simulink model "Task 2 – Battery Modeling"  (R2025b)
settings: Solver=ode23tb  StartTime=0.0  StopTime=35  RelTol=5e-3
model workspace (MAT data in the model file):
  Eng : object (value not decoded)
  Nmtr = 18.5
  SteerLim = 60
  TrackPoints = [-15 -12 -9 -6 -3 5.58745102111e-16 2.81978007367 5.36354042717 7.38228007367 8.67839071119 9.125 8.67839071119 ... (270 elements, 90x3)]
  Trans : object (value not decoded)
  Ts = 0.02
  VEH : object (value not decoded)
symbols that are objects in the model workspace (value not decoded): Eng, Trans, VEH
undefined symbols (not defined in the file or in its folder): BdyFrm, InertFrm
libraries: autolibsharedcoupling x11, simulink x9, sim3dlib x7, autolibutils x5, autolibshareddiff x5, sim3dautolib x3, vehdynlibtirecommon x3, sharedtransform x3, vehdynlibdriver x2, vehdynlibviscommon x2, vehdynlibtire x1, autolibmappedmotor x1
(part 2 of 4)

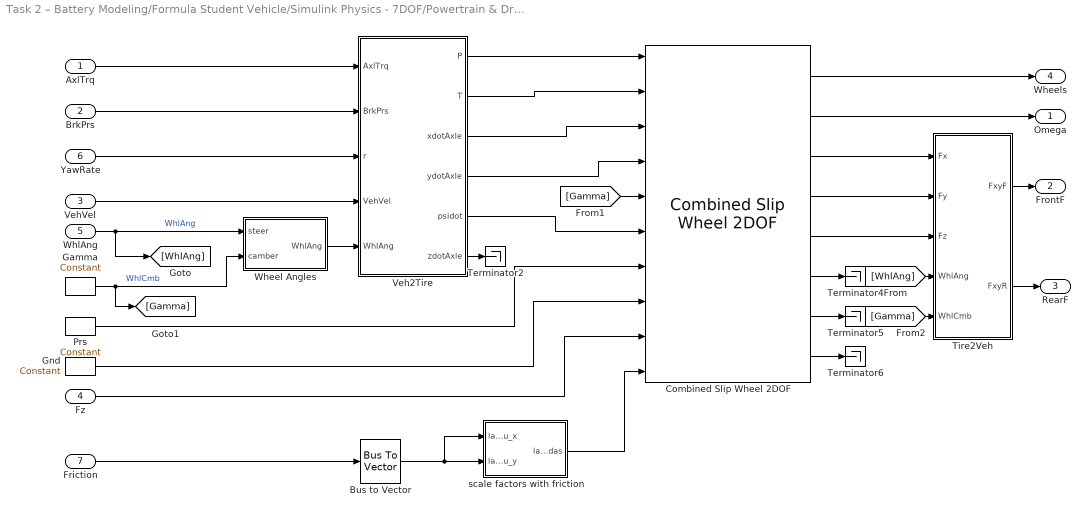
== system Task 2 – Battery Modeling/Formula Student Vehicle/Simulink Physics - 7DOF/Powertrain & Driveline/Brakes and Wheels ==
  AxlTrq : Inport
  BrkPrs : Inport  Port=2
  VehVel : Inport  Port=3
  Fz : Inport  Port=4  PortDimensions=4
  WhlAng : Inport  Port=5
  YawRate : Inport  Port=6
  Friction : Inport  Port=7
  Bus to Vector : BusToVector
  Combined Slip Wheel 2DOF : vehdynlibtire/Combined Slip Wheel 2DOF  tireType=External file  tireParamSet=skidpadtire.mat  vertType=None  plySteer=off  turnslip=off  BrakeType=Disc  mu_static=.3  mu_kinetic=.2  drum_abore=0.0508  drum_a=0.123  drum_c=0.212  drum_r=0.15  drum_theta1=0  drum_theta2=126  disk_abore=.05  Rm=.177  num_pads=2  brake_p_bpt=[1 11.4736842105263 21.9473684210526 32.4210526315789 42.8947368421053 53.3684210526316 63.8421052631579 74.3157894736842 84.7894736842105 95.2631578947368 105.736842105263 116.210526315789 126.684210526316 137.157894736842 147.631578947368 158.105263157895 168.578947368421 179.052631578947 189.526315789474 200]  brake_n_bpt=[0 52.6315789473684 105.263157894737 157.894736842105 210.526315789474 263.157894736842 315.789473684211 368.421052631579 421.052631578947 473.684210526316 526.315789473684 578.947368421053 631.578947368421 684.210526315789 736.842105263158 789.473684210526 842.105263157895 894.736842105263 947.368421052632 1000]  f_brake_t=[43.4900602404453 42.5056030554862 41.5350898940194 40.5780454442085 39.6340111501808 38.7025443887544 37.7832176914519 36.8756180088306 35.9793460143796 35.0940154454303 34.2192524787115 33.3546951383474 32.4999927342521 31.6548053290159 30.8188032315107 29.991666515561 29.1730845621415 28.362755623661 27.5603864089927 26.765691687993;498.991217495636 487.695866636631 476.560505099801 465.579679307235 454.748127933653 444.060772460445 433.51270824929 423.099196101319 412.81565427025 402.657650900201 392.620896861006 382.701238955775 372.894653477208 363.197240090814 353.605216024701 344.114910546964 334.722759712992 325.425301366216 316.219170376863 307.10109410434;954.492374750826 932.886130217776 911.585920305583 890.581313170261 869.862244717126 849.419000532136 829.242198807128 809.322774193808 789.651962526121 770.221286354971 751.0225412433 732.047782773203 713.289314220164 694.739674852612 676.391628817892 658.238154578366 640.272434863842 622.48784710877 604.877954344734 587.436496520688;1409.99353200602 1378.07639379892 1346.61133551136 1315.58294703329 1284.9763615006 1254.77722860383 1224.97168936497 1195.5463522863 1166.48827078199 1137.78492180974 1109.42418562559 1081.39432659063 1053.68397496312 1026.28210961441 999.178041611083 972.361398609768 945.822110014692 919.550392851325 893.536738312604 867.771898937035;1865.49468926121 1823.26665738007 1781.63675071715 1740.58458089631 1700.09047828407 1660.13545667552 1620.7011799228 1581.76993037878 1543.32457903786 1505.34855726451 1467.82583000789 1430.74087040806 1394.07863570608 1357.82454437621 1321.96445440427 1286.48464264117 1251.37178516554 1216.61293859388 1182.19552228048 1148.10730135338;2320.9958465164 2268.45692096121 2216.66216592293 2165.58621475934 2115.20459506754 2065.49368474721 2016.43067048064 1967.99350847127 1920.16088729373 1872.91219271928 1826.22747439018 1780.08741422549 1734.47329644903 1689.36697913801 1644.75086719747 1600.60788667257 1556.92146031639 1513.67548433643 1470.85430624835 1428.44270376973;2776.49700377159 2713.64718454235 2651.68758112871 2590.58784862237 2530.31871185102 2470.8519128189 2412.16016103848 2354.21708656376 2296.9971955496 2240.47582817405 2184.62911877248 2129.43395804292 2074.86795719199 2020.9094138998 1967.53727999066 1914.73113070398 1862.47113546724 1810.73803007899 1759.51309021622 1708.77810618608;3231.99816102678 3158.8374481235 3086.71299633449 3015.58948248539 2945.43282863449 2876.21014089059 2807.88965159632 2740.44066465625 2673.83350380547 2608.03946362882 2543.03076315477 2478.78050186034 2415.26261793494 2352.4518486616 2290.32369278385 2228.85437473538 2168.02081061809 2107.80057582154 2048.17187418409 1989.11350860242;3687.49931828197 3604.02771170464 3521.73841154027 3440.59111634842 3360.54694541796 3281.56836896228 3203.61914215416 3126.66424274874 3050.66981206134 2975.60309908359 2901.43240753707 2828.12704567777 2755.6572786779 2683.9942834234 2613.11010557704 2542.97761876678 2473.57048576894 2404.8631215641 2336.83065815196 2269.44891101877;4143.00047553716 4049.21797528579 3956.76382674606 3865.59275021144 3775.66106220143 3686.92659703397 3599.34863271199 3512.88782084123 3427.50612031721 3343.16673453836 3259.83405191936 3177.4735894952 3096.05193942085 3015.5367181852 2935.89651837023 2857.10086279818 2779.12016091979 2701.92566730665 2625.48944211983 2549.78431343512;4598.50163279235 4494.40823886693 4391.78924195184 4290.59438407447 4190.77517898491 4092.28482510566 3995.07812326983 3899.11139893372 3804.34242857308 3710.73036999313 3618.23569630166 3526.82013331263 3436.44660016381 3347.079152947 3258.68293116342 3171.22410682959 3084.66983607064 2998.98821304921 2914.1482260877 2830.11971585147;5054.00279004754 4939.59850244808 4826.81465715762 4715.59601793749 4605.88929576838 4497.64305317735 4390.80761382767 4285.3349770262 4181.17873682896 4078.2940054479 3976.63734068395 3876.16667713006 3776.84126090677 3678.62158770879 3581.46934395661 3485.34735086099 ...(+2764 chars)]  NOMPRES=78844.9  PRESMAX=99780  PRESMIN=45540  FNOMIN=866  FZMAX=1688  FZMIN=185  VXLOW=1  KPUMAX=0.165  KPUMIN=-0.179  ALPMAX=0.2338  ALPMIN=-0.2293  CAMMAX=0.0699  CAMMIN=-0.0699  LONGVL=10.23  FxRelFreqLwrLim=200*pi  FyRelFreqLwrLim=200*pi  MyRelFreqLwrLim=100*pi  omegao=0  UNLOADED_RADIUS=0.2667  WIDTH=0.2032  RIM_RADIUS=0.1651  ASPECT_RATIO=0.5  MASS=9.3  IYY=0.736  br=1e-3  GRAVITY=-9.81  zo=0  zdoto=0  BREFF=13.804  DREFF=1.08343  FREFF=0.16356  Q_RE0=0.9974  Q_V1=0.00077  Q_V2=9e-05  Q_FZ1=0  Q_FZ2=482.2  Q_FZ3=0  Q_FCX=0  Q_FCY=0  Q_FCY2=0  PFZ1=0.7098  VERTICAL_STIFFNESS=142605.8  VERTICAL_DAMPING=50  BOTTOM_OFFST=0.01  BOTTOM_STIFF=2000000  Q_CAM1=0  Q_CAM2=0  Q_CAM3=0  Q_FYS1=0  Q_FYS2=0  Q_FYS3=0  LONGITUDINAL_STIFFNESS=256665.8  LATERAL_STIFFNESS=128332.9  PCFX1=0.17504  PCFX2=0  PCFX3=0  PCFY1=-0.03642  PCFY2=-0.27821  PCFY3=0.85328  Q_RA1=0.671  Q_RA2=0.733  Q_RB1=1.059  Q_RB2=-1.1878  PCX1=1.33219  PDX1=2.49208  PDX2=-0.29183  PDX3=17.333  PEX1=-0.17111  PEX2=-0.4131  PEX3=0.02988  PEX4=0.49997  PKX1=71.453  PKX2=8.97121  PKX3=-0.45183  PHX1=-0.00015  PHX2=0.00067  PVX1=0.00734  PVX2=-0.07916  PPX1=-0.43509  PPX2=-0.99317  PPX3=-0.33222  PPX4=0.65659  RBX1=19.88  RBX2=18.46  RBX3=0.0011  RCX1=1.04033  REX1=0.04635  REX2=0.61362  RHX1=0.00055  QSX1=-0.00353  QSX2=1.0358  QSX3=-0.13483  QSX4=2.77124  QSX5=2.08896  QSX6=7.47056  QSX7=1.4241  QSX8=-1.49052  QSX9=0.04655  QSX10=2.8746  QSX11=2.56329  QSX12=0  QSX13=0  QSX14=0  PPMX1=0  PCY1=1.43572  PDY1=2.47082  PDY2=-0.32845  PDY3=9.99931  PEY1=-0.03742  PEY2=0.00966  PEY3=4.30184  PEY4=9.9963  PEY5=-9.44404  PKY1=-59.921  PKY2=3.17207  PKY3=1.4496  PKY4=3.23539  PKY5=9.99796  PKY6=-4.35202  PKY7=-0.97534  PHY1=0.00014  PHY2=-0.0004  PVY1=0.02954  PVY2=-0.00533  PVY3=0.29771  PVY4=0.37122  PPY1=0.47177  PPY2=1.18884  PPY3=-0.09605  PPY4=-0.06225  PPY5=-0.05092  RBY1=20.598  RBY2=18.246  RBY3=-0.00953  RBY4=-9.99975  RCY1=1.35742  REY1=1.68336  REY2=0.86596  RHY1=0.00563  RHY2=0.0134  RVY1=-0.02365  RVY2=0.15753  RVY3=9.95756  RVY4=40.921  RVY5=6.36739  RVY6=0.13517  QSY1=0.00702  QSY2=0  QSY3=0.00152  QSY4=9e-05  QSY5=0  QSY6=0  QSY7=0.9008  QSY8=-0.4089  QBZ1=8.10783  QBZ2=-2.90307  QBZ3=0.4997  QBZ4=0.11125  QBZ5=-0.19133  QBZ6=0  QBZ9=21.47  QBZ10=0.49977  QCZ1=1.82596  QDZ1=0.11638  QDZ2=-0.04294  QDZ3=1.71418  QDZ4=-9.64864  QDZ6=-0.01628  QDZ7=0.0224  QDZ8=-1.94566  QDZ9=-0.18492  QDZ10=6.61597  QDZ11=-5.13592  QEZ1=0.69467  QEZ2=-0.24253  QEZ3=-0.31384  QEZ4=-0.13439  QEZ5=0.10271  QHZ1=-0.00416  QHZ2=0.00812  QHZ3=-0.37901  QHZ4=-0.13948  PPZ1=-0.4408  PPZ2=0  SSZ1=-0.00091  SSZ2=-0.00496  SSZ3=0.73194  SSZ4=0.04083  PDXP1=0.4  PDXP2=0  PDXP3=0  PKYP1=1  PDYP1=0.4  PDYP2=0  PDYP3=0  PDYP4=0  PHYP1=1  PHYP2=0.15  PHYP3=0  PHYP4=-4  PECP1=0.5  PECP2=0  QDTP1=10  QCRP1=0.2  QCRP2=0.1  QBRP1=0.1  QDRP1=1  QDRP2=0  aMode=2
  Gamma : vehdynlibtirecommon/Constant  const=0  numWheels=4
  Gnd : vehdynlibtirecommon/Constant  const=0  numWheels=4
  Prs : vehdynlibtirecommon/Constant  const=2.4e5*1.1  numWheels=4
  Terminator{2,4..6} (4 alike) : Terminator
  Tire2Veh : Subsystem
  Veh2Tire : Subsystem
  Wheel Angles : Subsystem
  scale factors with friction : Subsystem  mask{numWheels=4}
      mask prompts: numWheels "Number of wheels"
  Omega : Outport
  FrontF : Outport  Port=2
  RearF : Outport  Port=3
  Wheels : Outport  Port=4
  wires:
  Gnd/1 -> Combined Slip Wheel 2DOF/8
  Combined Slip Wheel 2DOF/1 -> Wheels/1
  Combined Slip Wheel 2DOF/2 -> Omega/1
  Combined Slip Wheel 2DOF/7 -> Terminator5/1
  Combined Slip Wheel 2DOF/6 -> Terminator4/1
  Fz/1 -> Combined Slip Wheel 2DOF/9
  Veh2Tire/3(xdotAxle) -> Combined Slip Wheel 2DOF/3
  Combined Slip Wheel 2DOF/8 -> Terminator6/1
  Prs/1 -> Combined Slip Wheel 2DOF/7
  Veh2Tire/5(psidot) -> Combined Slip Wheel 2DOF/6
  Combined Slip Wheel 2DOF/3 -> Tire2Veh/1(Fx)
  Combined Slip Wheel 2DOF/4 -> Tire2Veh/2(Fy)
  Combined Slip Wheel 2DOF/5 -> Tire2Veh/3(Fz)
  WhlAng/1 -> [WhlAng], Wheel Angles/1(steer)  "WhlAng"
  Gamma/1 -> [Gamma], Wheel Angles/2(camber)  "WhlCmb"
  Tire2Veh/1(FxyF) -> FrontF/1
  Tire2Veh/2(FxyR) -> RearF/1
  Veh2Tire/2(T) -> Combined Slip Wheel 2DOF/2
  BrkPrs/1 -> Veh2Tire/2(BrkPrs)
  AxlTrq/1 -> Veh2Tire/1(AxlTrq)
  Wheel Angles/1(WhlAng) -> Veh2Tire/5(WhlAng)
  VehVel/1 -> Veh2Tire/4(VehVel)
  Veh2Tire/6(zdotAxle) -> Terminator2/1
  Veh2Tire/1(P) -> Combined Slip Wheel 2DOF/1
  Veh2Tire/4(ydotAxle) -> Combined Slip Wheel 2DOF/4
  YawRate/1 -> Veh2Tire/3(r)
  [WhlAng] -> Tire2Veh/4(WhlAng)
  [Gamma] -> Combined Slip Wheel 2DOF/5
  [Gamma] -> Tire2Veh/5(WhlCmb)
  Friction/1 -> Bus to Vector/1
  scale factors with friction/1(lambdas) -> Combined Slip Wheel 2DOF/10
  Bus to Vector/1 -> scale factors with friction/1(lamda_mu_x), scale factors with friction/2(lamda_mu_y)

== system Task 2 – Battery Modeling/Formula Student Vehicle/Simulink Physics - 7DOF/Powertrain & Driveline/Dual ==
  VehFdbk : Inport
  Dual Fz : Subsystem
  Dual V : Subsystem
  VehVel : Outport  VectorParamsAs1DForOutWhenUnconnected=off
  Fz : Outport  Port=2  VectorParamsAs1DForOutWhenUnconnected=off
  wires:
  Dual V/1(Out1) -> VehVel/1
  VehFdbk/1 -> Dual Fz/1(In1), Dual V/1(In1)
  Dual Fz/1(Out1) -> Fz/1

== system Task 2 – Battery Modeling/Formula Student Vehicle/Simulink Physics - 7DOF/Powertrain & Driveline/Final Drive ==
  Omega : Inport
  DrvShfTrq : Inport  Port=2
  All Wheel Drive : Subsystem  VariantControl=AWD
  Direct : Subsystem  VariantControl=Direct
  Front Wheel Drive : Subsystem  VariantControl=FWD
  Rear Wheel Drive : Subsystem  VariantControl=RWD
  AxlTrq : Outport  VectorParamsAs1DForOutWhenUnconnected=off
  AxlSpd : Outport  Port=2  VectorParamsAs1DForOutWhenUnconnected=off

== system Task 2 – Battery Modeling/Formula Student Vehicle/Simulink Physics - 7DOF/Powertrain & Driveline/Powertrain ==
  HndWhl : Inport
  Acc : Inport  Port=2
  GearCmd : Inport  Port=3
  r : Inport  Port=4
  AxlSpd : Inport  Port=5
  4EM Powertrain : Subsystem  VariantControl=EV4EM
  ICE Powertrain : Subsystem  VariantControl=ICE
  MtrTrq : Outport
  MtrSpd : Outport  Port=2
  TransGearCmd : Outport  Port=3
  TransGear : Outport  Port=4
  DrvShftTrq : Outport  Port=5

== system Task 2 – Battery Modeling/Visualization/3D Visualization/Enabled/3D Visualization ==
  VehFdbk : Inport
  Disabled : Subsystem  VariantControl=engine3D==1
  Ground Following : Subsystem  VariantControl=engine3D==4
  Physical Vehicle : Subsystem  VariantControl=engine3D==3
  Simulation 3D Vehicle : Subsystem  VariantControl=engine3D==2

== system Task 2 – Battery Modeling/Visualization/3D Visualization/Enabled/Cones ==
  Disabled : Subsystem  VariantControl=conesOn==0
  Enabled : Subsystem  VariantControl=conesOn==1

== system Task 2 – Battery Modeling/Formula Student Vehicle/Simulink Physics - 7DOF/Environment/Ground Feedback/Constant ==
  Friction : Inport
  Bus Creator : BusCreator  Inputs=4
  Bus Creator2 : BusCreator  Inputs=4
  Bus Creator3 : BusCreator  Inputs=2
  Constant1 : Constant  Value=zeros(4,1)
  Demux : Demux
  Demux1 : Demux
  Signal Specification : SignalSpecification  Unit=m
  Signal Specification1 : SignalSpecification  Unit=1
  Ground : Outport  VectorParamsAs1DForOutWhenUnconnected=off
  wires:
  Bus Creator3/1 -> Ground/1
  Signal Specification1/1 -> Demux1/1
  Friction/1 -> Signal Specification1/1
  Bus Creator2/1 -> Bus Creator3/2  "mu"
  Demux1/2 -> Bus Creator2/2  "mu_FR"
  Demux1/1 -> Bus Creator2/1  "mu_FL"
  Demux1/4 -> Bus Creator2/4  "mu_RR"
  Demux1/3 -> Bus Creator2/3  "mu_RL"
  Bus Creator/1 -> Bus Creator3/1  "z"
  Demux/2 -> Bus Creator/2  "G_FR_z"
  Demux/3 -> Bus Creator/3  "G_RL_z"
  Demux/1 -> Bus Creator/1  "G_FL_z"
  Demux/4 -> Bus Creator/4  "G_RR_z"
  Signal Specification/1 -> Demux/1
  Constant1/1 -> Signal Specification/1

== system Task 2 – Battery Modeling/Formula Student Vehicle/Simulink Physics - 7DOF/Powertrain & Driveline/Brakes and Wheels/Tire2Veh ==
  Fx : Inport
  Fy : Inport  Port=2
  Fz : Inport  Port=3
  WhlAng : Inport  Port=4
  WhlCmb : Inport  Port=5
  Demux : Demux  Outputs=[2,2]
  Demux1 : Demux  Outputs=[2,2]
  Math Function : Math  Operator=transpose  SignedPower=on
  Signal Specification : SignalSpecification  Unit=N
  Signal Specification1 : SignalSpecification  Unit=N
  Signal Specification2 : SignalSpecification  Dimensions=4
  Signal Specification3 : SignalSpecification  Dimensions=4
  Signal Specification4 : SignalSpecification  Dimensions=4
  Terminator : Terminator
  Vector Concatenate5 : Concatenate  Mode=Multidimensional array  ConcatenateDimension=2
  Vector Concatenate6 : Concatenate  Mode=Multidimensional array  ConcatenateDimension=2
  Vector Concatenate8 : Concatenate  NumInputs=3  Mode=Multidimensional array  ConcatenateDimension=2
  Wheel Angles : Subsystem
  Wheel to Body Transform : Subsystem
  FxyF : Outport
  FxyR : Outport  Port=2
  wires:
  Wheel Angles/1(Vehicle) -> Wheel to Body Transform/2(WheelAngles)
  Vector Concatenate5/1 -> Signal Specification1/1
  Demux/1 -> Vector Concatenate5/1
  Vector Concatenate8/1 -> Math Function/1
  Signal Specification1/1 -> FxyF/1
  Wheel to Body Transform/1(Fx) -> Demux/1
  Vector Concatenate6/1 -> Signal Specification/1
  Signal Specification4/1 -> Vector Concatenate8/3
  Demux1/2 -> Vector Concatenate6/2
  Wheel to Body Transform/2(Fy) -> Demux1/1
  Fy/1 -> Signal Specification3/1
  Math Function/1 -> Wheel to Body Transform/1(Forces)
  Wheel to Body Transform/3(Fz) -> Terminator/1
  Demux/2 -> Vector Concatenate6/1
  Signal Specification3/1 -> Vector Concatenate8/2
  Signal Specification2/1 -> Vector Concatenate8/1
  Demux1/1 -> Vector Concatenate5/2
  WhlAng/1 -> Wheel Angles/1(Front)
  Fx/1 -> Signal Specification2/1
  Fz/1 -> Signal Specification4/1
  Signal Specification/1 -> FxyR/1
  WhlCmb/1 -> Wheel Angles/2(Camber)

== system Task 2 – Battery Modeling/Formula Student Vehicle/Simulink Physics - 7DOF/Powertrain & Driveline/Brakes and Wheels/Veh2Tire ==
  AxlTrq : Inport
  BrkPrs : Inport  Port=2
  r : Inport  Port=3
  VehVel : Inport  Port=4
  WhlAng : Inport  Port=5
  Reshape3 : Reshape
  Reshape4 : Reshape
  Selector : Selector  InputPortWidth=1  IndexOptions=Index vector (dialog)  Indices=[1 1 1 1]  OutputSizes=1
  Unary Minus : UnaryMinus
  Wheel to Body Transform : Subsystem
  P : Outport  PortDimensions=4  VectorParamsAs1DForOutWhenUnconnected=off
  T : Outport  Port=2  VectorParamsAs1DForOutWhenUnconnected=off
  xdotAxle : Outport  Port=3  PortDimensions=4  VectorParamsAs1DForOutWhenUnconnected=off
  ydotAxle : Outport  Port=4  PortDimensions=4  VectorParamsAs1DForOutWhenUnconnected=off
  psidot : Outport  Port=5  PortDimensions=4  VectorParamsAs1DForOutWhenUnconnected=off
  zdotAxle : Outport  Port=6  VectorParamsAs1DForOutWhenUnconnected=off
  wires:
  BrkPrs/1 -> Reshape3/1
  AxlTrq/1 -> Reshape4/1
  Wheel to Body Transform/1(xdotWheel) -> xdotAxle/1  "Vx"
  Wheel to Body Transform/2(ydotWheel) -> ydotAxle/1  "Vy"
  r/1 -> Unary Minus/1
  Reshape4/1 -> T/1
  VehVel/1 -> Wheel to Body Transform/1(VelVeh)
  Wheel to Body Transform/3(zdotWheel) -> zdotAxle/1  "Vz"
  Unary Minus/1 -> Selector/1
  Reshape3/1 -> P/1
  WhlAng/1 -> Wheel to Body Transform/2(WhlAng)
  Selector/1 -> psidot/1

== system Task 2 – Battery Modeling/Formula Student Vehicle/Simulink Physics - 7DOF/Powertrain & Driveline/Brakes and Wheels/Wheel Angles ==
  steer : Inport
  camber : Inport  Port=2
  Add1 : Sum
  Add2 : Sum
  Constant1 : Constant  Value=pi
  Constant2 : Constant  Value=[pi;0;pi;0].*0+[0;pi;0;pi].*0
  Constant3 : Constant  Value=ones(1,4).*0
  Reshape : Reshape  OutputDimensionality=Row vector (2-D)
  Reshape1 : Reshape  OutputDimensionality=Row vector (2-D)
  Reshape2 : Reshape  OutputDimensionality=Row vector (2-D)
  Vector Concatenate3 : Concatenate  NumInputs=3  Mode=Multidimensional array
  WhlAng : Outport  VectorParamsAs1DForOutWhenUnconnected=off
  wires:
  Constant1/1 -> Add2/2
  Add2/1 -> Reshape1/1
  Add1/1 -> Reshape/1
  Reshape2/1 -> Vector Concatenate3/2
  Reshape1/1 -> Vector Concatenate3/1
  Constant3/1 -> Reshape2/1
  camber/1 -> Add2/1
  steer/1 -> Add1/1
  Reshape/1 -> Vector Concatenate3/3
  Vector Concatenate3/1 -> WhlAng/1
  Constant2/1 -> Add1/2

== system Task 2 – Battery Modeling/Formula Student Vehicle/Simulink Physics - 7DOF/Powertrain & Driveline/Brakes and Wheels/scale factors with friction ==
  lamda_mu_x : Inport
  lamda_mu_y : Inport  Port=2
  0 : Constant  Value=[zeros(1,numWheels)]  VectorParams1D=off
  Reshape : Reshape  OutputDimensionality=Row vector (2-D)  OutputDimensions=[1,numWheels]
  Reshape1 : Reshape  OutputDimensionality=Row vector (2-D)  OutputDimensions=[1,numWheels]
  Signal Specification3 : SignalSpecification  Unit=1
  Vector Concatenate : Concatenate  NumInputs=5  Mode=Multidimensional array
  ones : Constant  Value=[ones(23,numWheels)]  VectorParams1D=off
  ones2 : Constant  Value=ones(1,numWheels)  VectorParams1D=off
  lambdas : Outport  Unit=1  VectorParamsAs1DForOutWhenUnconnected=off
  wires:
  lamda_mu_y/1 -> Reshape1/1
  lamda_mu_x/1 -> Reshape/1
  ones2/1 -> Vector Concatenate/1  "lambda_Fz0"
  Vector Concatenate/1 -> Signal Specification3/1
  ones/1 -> Vector Concatenate/5
  0/1 -> Vector Concatenate/4  "lamda_mu_V"
  Reshape1/1 -> Vector Concatenate/3
  Reshape/1 -> Vector Concatenate/2
  Signal Specification3/1 -> lambdas/1

== system Task 2 – Battery Modeling/Formula Student Vehicle/Simulink Physics - 7DOF/Powertrain & Driveline/Dual/Dual Fz ==
  In1 : Inport
  Add : Sum
  Bus Selector6 : BusSelector  OutputSignals=BdyFrm.Forces.Tires.FrntTires.Lft.Fz,BdyFrm.Forces.Tires.FrntTires.Rght.Fz,BdyFrm.Forces.Tires.RearTires.Lft.Fz,BdyFrm.Forces.Tires.RearTires.Rght.Fz
  Cont LPF : autolibutils/Cont LPF  wc=100*2*pi  AbsoluteTolerance=auto  aMode=2
  Saturation : Saturate  UpperLimit=10e3  LowerLimit=100  ZeroCross=off
  Unsprung Mass : Constant  Value="[5 5  5 5].*9.81"
  Vector Concatenate : Concatenate  NumInputs=4
  Out1 : Outport  VectorParamsAs1DForOutWhenUnconnected=off
  wires:
  Saturation/1 -> Cont LPF/1
  Cont LPF/1 -> Add/1
  Vector Concatenate/1 -> Saturation/1
  Bus Selector6/2 -> Vector Concatenate/2  "<Fz>"
  Bus Selector6/1 -> Vector Concatenate/1  "<Fz>"
  Bus Selector6/3 -> Vector Concatenate/3  "<Fz>"
  Bus Selector6/4 -> Vector Concatenate/4  "<Fz>"
  Add/1 -> Out1/1
  Unsprung Mass/1 -> Add/2
  In1/1 -> Bus Selector6/1

== system Task 2 – Battery Modeling/Formula Student Vehicle/Simulink Physics - 7DOF/Powertrain & Driveline/Dual/Dual V ==
  In1 : Inport
  Bus Selector1 : BusSelector  OutputSignals=BdyFrm.FrntAxl.Lft.Vel.xdot,BdyFrm.FrntAxl.Lft.Vel.ydot,BdyFrm.FrntAxl.Lft.Vel.zdot  OutputAsBus=on
  Bus Selector2 : BusSelector  OutputSignals=BdyFrm.FrntAxl.Rght.Vel.xdot,BdyFrm.FrntAxl.Rght.Vel.ydot,BdyFrm.FrntAxl.Rght.Vel.zdot  OutputAsBus=on
  Bus Selector4 : BusSelector  OutputSignals=BdyFrm.RearAxl.Lft.Vel.xdot,BdyFrm.RearAxl.Lft.Vel.ydot,BdyFrm.RearAxl.Lft.Vel.zdot  OutputAsBus=on
  Bus Selector5 : BusSelector  OutputSignals=BdyFrm.RearAxl.Rght.Vel.xdot,BdyFrm.RearAxl.Rght.Vel.ydot,BdyFrm.RearAxl.Rght.Vel.zdot  OutputAsBus=on
  Bus to Vector{5..8} (4 alike) : BusToVector
  Vector Concatenate2 : Concatenate  NumInputs=4  Mode=Multidimensional array  ConcatenateDimension=2
  Out1 : Outport  VectorParamsAs1DForOutWhenUnconnected=off
  wires:
  Bus to Vector6/1 -> Vector Concatenate2/2
  Bus Selector2/1 -> Bus to Vector6/1
  Bus to Vector8/1 -> Vector Concatenate2/4
  Bus Selector4/1 -> Bus to Vector7/1
  Bus to Vector5/1 -> Vector Concatenate2/1
  Bus Selector1/1 -> Bus to Vector5/1
  Bus Selector5/1 -> Bus to Vector8/1
  Bus to Vector7/1 -> Vector Concatenate2/3
  Vector Concatenate2/1 -> Out1/1
  In1/1 -> Bus Selector1/1, Bus Selector2/1, Bus Selector4/1, Bus Selector5/1

== system Task 2 – Battery Modeling/Formula Student Vehicle/Simulink Physics - 7DOF/Powertrain & Driveline/Final Drive/All Wheel Drive ==
  DrvShfTrq : Inport
  Omega : Inport  Port=2
  Demux1 : Demux  Outputs=2
  Demux2 : Demux  Outputs=2
  Demux3 : Demux  Outputs=2
  Limited Slip Differential : autolibshareddiff/Limited Slip Differential  DiffEffModelPopup=Constant  InterpMethod=Linear point-slope  extTamb=off  shaftSwitchMask=To the left of center-line  Ndiff=4  Jd=.1  bd=1e-3  Jw1=.1  bw1=1e-3  Jw2=.1  bw2=1e-3  omegaw1o=0  omegaw2o=0  eta=1  eta_tbl=reshape([0.64 0.76 0.8 0.81 0.83 0.84 0.84 0.56 0.73 0.78 0.8 0.83 0.84 0.84 0.54 0.71 0.77 0.8 0.82 0.84 0.84 0.53 0.71 0.77 0.8 0.83 0.84 0.84 0.51 0.71 0.77 0.8 0.83 0.84 0.85 0.52 0.7 0.77 0.8 0.83 0.84 0.85 0.51 0.71 0.76 0.79 0.83 0.84 0.85 0.5 0.69 0.76 0.79 0.82 0.84 0.85 0.45 0.68 0.75 0.78 0.82 0.84 0.85 0.43 0.67 0.74 0.78 0.81 0.83 0.84 0.38 0.63 0.71 0.75 0.8 0.82 0.83 0.81 0.86 0.88 0.89 0.89 0.89 0.9 0.77 0.85 0.87 0.88 0.89 0.9 0.9 0.72 0.82 0.86 0.87 0.88 0.89 0.9 0.68 0.8 0.84 0.86 0.88 0.89 0.89 0.67 0.8 0.84 0.86 0.88 0.89 0.9 0.67 0.8 0.84 0.86 0.88 0.89 0.9 0.65 0.8 0.84 0.86 0.88 0.89 0.9 0.64 0.79 0.83 0.86 0.88 0.89 0.9 0.63 0.78 0.83 0.86 0.88 0.89 0.9 0.59 0.76 0.82 0.85 0.87 0.89 0.9 0.53 0.73 0.8 0.83 0.86 0.88 0.89], 7, 11, 2)  Trq_bpts=[25, 50, 75, 100, 150, 200, 250]  omega_bpts=[52.4 78.5 105 131 157 183 209 262 314 419 524]  Temp_bpts=[290 358]  Tamb=297.15  couplingType=Pre-loaded ideal clutch  Ndisks=4  Reff=.20  Fc=500  muc=[.16 0.13 0.115 0.11 0.105 0.1025 0.10125]  dw=[0 10 20 40 60 80 100]  Tdw=[-100, -90, -50, -5, 0, 5, 50, 90, 100]  dwT=[-200, -175, -100, - 50, 0, 50, 100, 175, 200]  TTin=[-200 -175 -100 - 50 0 50 100 175 200]  Tin=[-200 -175 -100 - 50 0 50 100 175 200]  tauC=.01  IdealInterpMethod=Linear point-slope  IdealExtrapMethod=Clip  TdwInterpMethod=Linear point-slope  TdwExtrapMethod=Clip  TTinInterpMethod=Linear point-slope  TTinExtrapMethod=Clip  maxAbsSpd=5e3  aMode=2
      settings: LibrarySourceBlock=vdynlib/Powertrain/Drivetrain/Final Drive Unit/Limited Slip Differential
  Open Differential : autolibshareddiff/Open Differential  DiffEffModelPopup=Constant  InterpMethod=Linear point-slope  extTamb=off  shaftSwitchMask=To the left of center-line  Ndiff=4  Jd=.1  bd=1e-3  Jw1=.1  bw1=1e-3  Jw2=.1  bw2=1e-3  omegaw1o=0  omegaw2o=0  eta=1  eta_tbl=reshape([0.64 0.76 0.8 0.81 0.83 0.84 0.84 0.56 0.73 0.78 0.8 0.83 0.84 0.84 0.54 0.71 0.77 0.8 0.82 0.84 0.84 0.53 0.71 0.77 0.8 0.83 0.84 0.84 0.51 0.71 0.77 0.8 0.83 0.84 0.85 0.52 0.7 0.77 0.8 0.83 0.84 0.85 0.51 0.71 0.76 0.79 0.83 0.84 0.85 0.5 0.69 0.76 0.79 0.82 0.84 0.85 0.45 0.68 0.75 0.78 0.82 0.84 0.85 0.43 0.67 0.74 0.78 0.81 0.83 0.84 0.38 0.63 0.71 0.75 0.8 0.82 0.83 0.81 0.86 0.88 0.89 0.89 0.89 0.9 0.77 0.85 0.87 0.88 0.89 0.9 0.9 0.72 0.82 0.86 0.87 0.88 0.89 0.9 0.68 0.8 0.84 0.86 0.88 0.89 0.89 0.67 0.8 0.84 0.86 0.88 0.89 0.9 0.67 0.8 0.84 0.86 0.88 0.89 0.9 0.65 0.8 0.84 0.86 0.88 0.89 0.9 0.64 0.79 0.83 0.86 0.88 0.89 0.9 0.63 0.78 0.83 0.86 0.88 0.89 0.9 0.59 0.76 0.82 0.85 0.87 0.89 0.9 0.53 0.73 0.8 0.83 0.86 0.88 0.89], 7, 11, 2)  Trq_bpts=[25, 50, 75, 100, 150, 200, 250]  omega_bpts=[52.4 78.5 105 131 157 183 209 262 314 419 524]  Temp_bpts=[290 358]  Tamb=297.15  maxAbsSpd=5e3  aMode=2
      settings: LibrarySourceBlock=vdynlib/Powertrain/Drivetrain/Final Drive Unit/Open Differential
  Terminator : Terminator
  Terminator1 : Terminator
  Terminator2 : Terminator
  Torsional Compliance{,1..3} (4 alike) : autolibsharedcoupling/Torsional Compliance  port_config=Simulink  extInfo=off  k=5e3  b=50  theta_o=0  domega_o=0  omega_c=150  blkID=0  aMode=2
      settings: LibrarySourceBlock=vdynlib/Powertrain/Drivetrain/Couplings/Torsional Compliance
  Torsional Compliance4 : autolibsharedcoupling/Torsional Compliance  port_config=Simulink  extInfo=off  k=1e4  b=1e2  theta_o=0  domega_o=0  omega_c=3000  blkID=0  aMode=2
      settings: LibrarySourceBlock=vdynlib/Powertrain/Drivetrain/Couplings/Torsional Compliance
  Torsional Compliance5 : autolibsharedcoupling/Torsional Compliance  port_config=Simulink  extInfo=off  k=1e4  b=1e2  theta_o=0  domega_o=0  omega_c=3000  blkID=0  aMode=2
      settings: LibrarySourceBlock=vdynlib/Powertrain/Drivetrain/Couplings/Torsional Compliance
  Transfer Case : autolibshareddiff/Transfer Case  DiffEffModelPopup=Constant  InterpMethod=Linear point-slope  extTamb=off  TrqSplitRatioMode=off  SpdLockMode=off  shaftSwitchMask=To the left of center-line  Ndiff=1  Jd=.1  bd=1e-3  Jw1=.1  bw1=1e-3  Jw2=.1  bw2=1e-3  omegaw1o=0  omegaw2o=0  eta=1  eta_tbl=reshape([0.64 0.76 0.8 0.81 0.83 0.84 0.84 0.56 0.73 0.78 0.8 0.83 0.84 0.84 0.54 0.71 0.77 0.8 0.82 0.84 0.84 0.53 0.71 0.77 0.8 0.83 0.84 0.84 0.51 0.71 0.77 0.8 0.83 0.84 0.85 0.52 0.7 0.77 0.8 0.83 0.84 0.85 0.51 0.71 0.76 0.79 0.83 0.84 0.85 0.5 0.69 0.76 0.79 0.82 0.84 0.85 0.45 0.68 0.75 0.78 0.82 0.84 0.85 0.43 0.67 0.74 0.78 0.81 0.83 0.84 0.38 0.63 0.71 0.75 0.8 0.82 0.83 0.81 0.86 0.88 0.89 0.89 0.89 0.9 0.77 0.85 0.87 0.88 0.89 0.9 0.9 0.72 0.82 0.86 0.87 0.88 0.89 0.9 0.68 0.8 0.84 0.86 0.88 0.89 0.89 0.67 0.8 0.84 0.86 0.88 0.89 0.9 0.67 0.8 0.84 0.86 0.88 0.89 0.9 0.65 0.8 0.84 0.86 0.88 0.89 0.9 0.64 0.79 0.83 0.86 0.88 0.89 0.9 0.63 0.78 0.83 0.86 0.88 0.89 0.9 0.59 0.76 0.82 0.85 0.87 0.89 0.9 0.53 0.73 0.8 0.83 0.86 0.88 0.89], 7, 11, 2)  Trq_bpts=[25, 50, 75, 100, 150, 200, 250]  omega_bpts=[52.4 78.5 105 131 157 183 209 262 314 419 524]  Temp_bpts=[290 358]  Tamb=297.15  maxAbsSpd=5e3  aMode=2  TrqSplitRatio=0.5  SpdLock=0
      settings: LibrarySourceBlock=vdynlib/Powertrain/Drivetrain/Final Drive Unit/Transfer Case
  Vector Concatenate : Concatenate  NumInputs=4
  AxlTrq : Outport  VectorParamsAs1DForOutWhenUnconnected=off
  AxlSpd : Outport  Port=2  VectorParamsAs1DForOutWhenUnconnected=off
  wires:
  Torsional Compliance2/1 -> Limited Slip Differential/2
  Torsional Compliance3/1 -> Limited Slip Differential/3
  Limited Slip Differential/4 -> Torsional Compliance3/1
  Limited Slip Differential/1 -> Terminator/1
  Demux1/1 -> Torsional Compliance4/2
  Limited Slip Differential/3 -> Torsional Compliance2/1
  Transfer Case/1 -> Terminator1/1
  Transfer Case/2 -> AxlSpd/1
  DrvShfTrq/1 -> Transfer Case/1
  Torsional Compliance3/2 -> Vector Concatenate/4  "T_RR"
  Vector Concatenate/1 -> AxlTrq/1
  Transfer Case/3 -> Torsional Compliance/2
  Transfer Case/4 -> Torsional Compliance1/2
  Torsional Compliance/1 -> Open Differential/1
  Open Differential/2 -> Torsional Compliance/1
  Limited Slip Differential/2 -> Torsional Compliance1/1
  Torsional Compliance1/2 -> Transfer Case/3
  Torsional Compliance/2 -> Transfer Case/2
  Torsional Compliance1/1 -> Limited Slip Differential/1
  Omega/1 -> Demux2/1
  Demux2/1 -> Demux1/1
  Demux2/2 -> Demux3/1
  Demux1/2 -> Torsional Compliance5/2
  Open Differential/3 -> Torsional Compliance4/1
  Open Differential/4 -> Torsional Compliance5/1
  Demux3/1 -> Torsional Compliance2/2
  Demux3/2 -> Torsional Compliance3/2
  Open Differential/1 -> Terminator2/1
  Torsional Compliance4/1 -> Open Differential/2
  Torsional Compliance5/1 -> Open Differential/3
  Torsional Compliance4/2 -> Vector Concatenate/1  "T_FL"
  Torsional Compliance5/2 -> Vector Concatenate/2  "T_FR"
  Torsional Compliance2/2 -> Vector Concatenate/3  "T_RL"

== system Task 2 – Battery Modeling/Formula Student Vehicle/Simulink Physics - 7DOF/Powertrain & Driveline/Final Drive/Direct ==
  DrvShfTrq : Inport
  Omega : Inport  Port=2
  AxlTrq : Outport  VectorParamsAs1DForOutWhenUnconnected=off
  AxlSpd : Outport  Port=2  VectorParamsAs1DForOutWhenUnconnected=off
  wires:
  Omega/1 -> AxlSpd/1
  DrvShfTrq/1 -> AxlTrq/1

== system Task 2 – Battery Modeling/Formula Student Vehicle/Simulink Physics - 7DOF/Powertrain & Driveline/Final Drive/Front Wheel Drive ==
  DrvShfTrq : Inport
  Omega : Inport  Port=2
  Demux : Demux  Outputs=[2,2]
  Demux1 : Demux  Outputs=2
  Ground : Ground
  Ground1 : Ground
  Limited Slip Differential : autolibshareddiff/Limited Slip Differential  DiffEffModelPopup=Constant  InterpMethod=Linear point-slope  extTamb=off  shaftSwitchMask=To the left of center-line  Ndiff=Trans.FinalDrive  Jd=.08  bd=1e-3  Jw1=.05  bw1=1e-3  Jw2=.05  bw2=1e-3  omegaw1o=0  omegaw2o=0  eta=1  eta_tbl=reshape([0.64 0.76 0.8 0.81 0.83 0.84 0.84 0.56 0.73 0.78 0.8 0.83 0.84 0.84 0.54 0.71 0.77 0.8 0.82 0.84 0.84 0.53 0.71 0.77 0.8 0.83 0.84 0.84 0.51 0.71 0.77 0.8 0.83 0.84 0.85 0.52 0.7 0.77 0.8 0.83 0.84 0.85 0.51 0.71 0.76 0.79 0.83 0.84 0.85 0.5 0.69 0.76 0.79 0.82 0.84 0.85 0.45 0.68 0.75 0.78 0.82 0.84 0.85 0.43 0.67 0.74 0.78 0.81 0.83 0.84 0.38 0.63 0.71 0.75 0.8 0.82 0.83 0.81 0.86 0.88 0.89 0.89 0.89 0.9 0.77 0.85 0.87 0.88 0.89 0.9 0.9 0.72 0.82 0.86 0.87 0.88 0.89 0.9 0.68 0.8 0.84 0.86 0.88 0.89 0.89 0.67 0.8 0.84 0.86 0.88 0.89 0.9 0.67 0.8 0.84 0.86 0.88 0.89 0.9 0.65 0.8 0.84 0.86 0.88 0.89 0.9 0.64 0.79 0.83 0.86 0.88 0.89 0.9 0.63 0.78 0.83 0.86 0.88 0.89 0.9 0.59 0.76 0.82 0.85 0.87 0.89 0.9 0.53 0.73 0.8 0.83 0.86 0.88 0.89], 7, 11, 2)  Trq_bpts=[25, 50, 75, 100, 150, 200, 250]  omega_bpts=[52.4 78.5 105 131 157 183 209 262 314 419 524]  Temp_bpts=[290 358]  Tamb=297.15  couplingType=Pre-loaded ideal clutch  Ndisks=8  Reff=.08  Fc=1000  muc=[.16 0.13 0.115 0.11 0.105 0.1025 0.10125 .10125]  dw=[0 10 20 40 60 80 100 1000]  Tdw=[-100, -90, -50, -5, 0, 5, 50, 90, 100]  dwT=[-200, -175, -100, - 50, 0, 50, 100, 175, 200]  TTin=[-200 -175 -100 - 50 0 50 100 175 200]  Tin=[-200 -175 -100 - 50 0 50 100 175 200]  tauC=.04  IdealInterpMethod=Linear point-slope  IdealExtrapMethod=Linear  TdwInterpMethod=Flat  TdwExtrapMethod=Clip  TTinInterpMethod=Flat  TTinExtrapMethod=Clip  maxAbsSpd=5e3  aMode=2
      settings: LibrarySourceBlock=vdynlib/Powertrain/Drivetrain/Final Drive Unit/Limited Slip Differential
  Terminator : Terminator
  Terminator1 : Terminator
  Torsional Compliance1 : autolibsharedcoupling/Torsional Compliance  port_config=Simulink  extInfo=off  k=3e5  b=50  theta_o=0  domega_o=0  omega_c=150  blkID=0  aMode=2
      settings: LibrarySourceBlock=vdynlib/Powertrain/Drivetrain/Couplings/Torsional Compliance
  Torsional Compliance2 : autolibsharedcoupling/Torsional Compliance  port_config=Simulink  extInfo=off  k=3e5  b=50  theta_o=0  domega_o=0  omega_c=150  blkID=0  aMode=2
      settings: LibrarySourceBlock=vdynlib/Powertrain/Drivetrain/Couplings/Torsional Compliance
  Vector Concatenate : Concatenate  NumInputs=4
  AxlTrq : Outport  VectorParamsAs1DForOutWhenUnconnected=off
  AxlSpd : Outport  Port=2  VectorParamsAs1DForOutWhenUnconnected=off
  wires:
  Limited Slip Differential/3 -> Torsional Compliance2/1
  Demux1/1 -> Torsional Compliance2/2
  Limited Slip Differential/1 -> Terminator/1
  DrvShfTrq/1 -> Limited Slip Differential/1
  Limited Slip Differential/2 -> AxlSpd/1
  Limited Slip Differential/4 -> Torsional Compliance1/1
  Demux1/2 -> Torsional Compliance1/2
  Demux/1 -> Demux1/1
  Torsional Compliance1/1 -> Limited Slip Differential/3
  Torsional Compliance2/1 -> Limited Slip Differential/2
  Demux/2 -> Terminator1/1
  Ground/1 -> Vector Concatenate/4  "T_RR"
  Torsional Compliance1/2 -> Vector Concatenate/2  "T_FR"
  Ground1/1 -> Vector Concatenate/3  "T_RL"
  Torsional Compliance2/2 -> Vector Concatenate/1  "T_FL"
  Omega/1 -> Demux/1
  Vector Concatenate/1 -> AxlTrq/1

== system Task 2 – Battery Modeling/Formula Student Vehicle/Simulink Physics - 7DOF/Powertrain & Driveline/Final Drive/Rear Wheel Drive ==
  DrvShfTrq : Inport
  Omega : Inport  Port=2
  Demux : Demux  Outputs=[2,2]
  Demux1 : Demux  Outputs=2
  Ground : Ground
  Ground1 : Ground
  Limited Slip Differential : autolibshareddiff/Limited Slip Differential  DiffEffModelPopup=Constant  InterpMethod=Linear point-slope  extTamb=off  shaftSwitchMask=To the left of center-line  Ndiff=Trans.FinalDrive  Jd=.08  bd=1e-3  Jw1=.01  bw1=1e-3  Jw2=.01  bw2=1e-3  omegaw1o=0  omegaw2o=0  eta=1  eta_tbl=reshape([0.64 0.76 0.8 0.81 0.83 0.84 0.84 0.56 0.73 0.78 0.8 0.83 0.84 0.84 0.54 0.71 0.77 0.8 0.82 0.84 0.84 0.53 0.71 0.77 0.8 0.83 0.84 0.84 0.51 0.71 0.77 0.8 0.83 0.84 0.85 0.52 0.7 0.77 0.8 0.83 0.84 0.85 0.51 0.71 0.76 0.79 0.83 0.84 0.85 0.5 0.69 0.76 0.79 0.82 0.84 0.85 0.45 0.68 0.75 0.78 0.82 0.84 0.85 0.43 0.67 0.74 0.78 0.81 0.83 0.84 0.38 0.63 0.71 0.75 0.8 0.82 0.83 0.81 0.86 0.88 0.89 0.89 0.89 0.9 0.77 0.85 0.87 0.88 0.89 0.9 0.9 0.72 0.82 0.86 0.87 0.88 0.89 0.9 0.68 0.8 0.84 0.86 0.88 0.89 0.89 0.67 0.8 0.84 0.86 0.88 0.89 0.9 0.67 0.8 0.84 0.86 0.88 0.89 0.9 0.65 0.8 0.84 0.86 0.88 0.89 0.9 0.64 0.79 0.83 0.86 0.88 0.89 0.9 0.63 0.78 0.83 0.86 0.88 0.89 0.9 0.59 0.76 0.82 0.85 0.87 0.89 0.9 0.53 0.73 0.8 0.83 0.86 0.88 0.89], 7, 11, 2)  Trq_bpts=[25, 50, 75, 100, 150, 200, 250]  omega_bpts=[52.4 78.5 105 131 157 183 209 262 314 419 524]  Temp_bpts=[290 358]  Tamb=297.15  couplingType=Pre-loaded ideal clutch  Ndisks=4  Reff=.08  Fc=1000  muc=[.16 0.13 0.115 0.11 0.105 0.1025 0.10125 .10125]  dw=[0 10 20 40 60 80 100 1000]  Tdw=[-100, -90, -50, -5, 0, 5, 50, 90, 100]  dwT=[-200, -175, -100, - 50, 0, 50, 100, 175, 200]  TTin=[-200 -175 -100 - 50 0 50 100 175 200]  Tin=[-200 -175 -100 - 50 0 50 100 175 200]  tauC=.04  IdealInterpMethod=Linear point-slope  IdealExtrapMethod=Linear  TdwInterpMethod=Flat  TdwExtrapMethod=Clip  TTinInterpMethod=Flat  TTinExtrapMethod=Clip  maxAbsSpd=5e3  aMode=2
      settings: LibrarySourceBlock=vdynlib/Powertrain/Drivetrain/Final Drive Unit/Limited Slip Differential
  Terminator : Terminator
  Terminator1 : Terminator
  Torsional Compliance : autolibsharedcoupling/Torsional Compliance  port_config=Simulink  extInfo=off  k=5e3  b=50  theta_o=0  domega_o=0  omega_c=600  blkID=0  aMode=2
      settings: LibrarySourceBlock=vdynlib/Powertrain/Drivetrain/Couplings/Torsional Compliance
  Torsional Compliance1 : autolibsharedcoupling/Torsional Compliance  port_config=Simulink  extInfo=off  k=5e3  b=50  theta_o=0  domega_o=0  omega_c=150  blkID=0  aMode=2
      settings: LibrarySourceBlock=vdynlib/Powertrain/Drivetrain/Couplings/Torsional Compliance
  Vector Concatenate : Concatenate  NumInputs=4
  AxlTrq : Outport  VectorParamsAs1DForOutWhenUnconnected=off
  AxlSpd : Outport  Port=2  VectorParamsAs1DForOutWhenUnconnected=off
  wires:
  Torsional Compliance/1 -> Limited Slip Differential/2
  Torsional Compliance1/1 -> Limited Slip Differential/3
  Demux/2 -> Demux1/1
  Demux1/2 -> Torsional Compliance1/2
  Limited Slip Differential/4 -> Torsional Compliance1/1
  Limited Slip Differential/2 -> AxlSpd/1
  DrvShfTrq/1 -> Limited Slip Differential/1
  Limited Slip Differential/1 -> Terminator/1
  Demux1/1 -> Torsional Compliance/2
  Limited Slip Differential/3 -> Torsional Compliance/1
  Demux/1 -> Terminator1/1
  Omega/1 -> Demux/1
  Torsional Compliance1/2 -> Vector Concatenate/4  "T_RR"
  Ground/1 -> Vector Concatenate/2  "T_FR"
  Ground1/1 -> Vector Concatenate/1  "T_FL"
  Torsional Compliance/2 -> Vector Concatenate/3  "T_RL"
  Vector Concatenate/1 -> AxlTrq/1

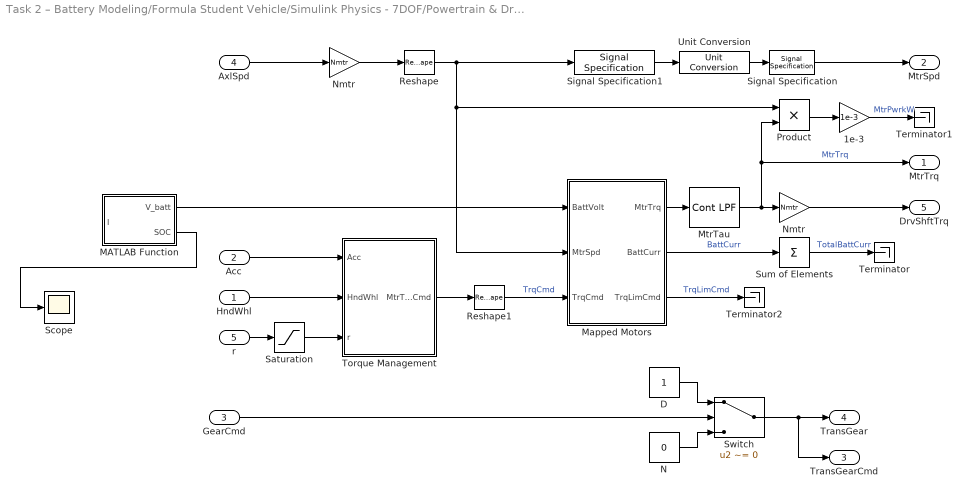
== system Task 2 – Battery Modeling/Formula Student Vehicle/Simulink Physics - 7DOF/Powertrain & Driveline/Powertrain/4EM Powertrain ==
  HndWhl : Inport
  Acc : Inport  Port=2
  GearCmd : Inport  Port=3
  AxlSpd : Inport  Port=4
  r : Inport  Port=5
  1e-3 : Gain  Gain=1e-3
  D : Constant
  MATLAB Function : MATLAB Function  TreatAsAtomicUnit=on
  Mapped Motors : Subsystem
  MtrTau : autolibutils/Cont LPF  wc=200*pi  AbsoluteTolerance=auto  aMode=2
  "N " : Constant  Value=0
  Nmtr : Gain  Gain=Nmtr
  "Nmtr " : Gain  Gain=Nmtr
  Product : Product
  Reshape : Reshape
  Reshape1 : Reshape
  Saturation : Saturate  UpperLimit=500*pi/180  LowerLimit=-500*pi/180  ZeroCross=off
  Scope : Scope
      settings: ActiveDisplayYMinimum=0.90578719526087947  ActiveDisplayYMaximum=1.09626338573707
  Signal Specification : SignalSpecification  Unit=rpm
  Signal Specification1 : SignalSpecification  Unit=rad/s
  Sum of Elements : Sum  Inputs=+
  Switch : Switch  Criteria=u2 ~= 0  ZeroCross=off  SaturateOnIntegerOverflow=off  InputSameDT=off
  Terminator : Terminator
  Terminator1 : Terminator
  Terminator2 : Terminator
  Torque Management : MATLAB Function  TreatAsAtomicUnit=on
  Unit Conversion : UnitConversion
  MtrTrq : Outport  VectorParamsAs1DForOutWhenUnconnected=off
  MtrSpd : Outport  Port=2  VectorParamsAs1DForOutWhenUnconnected=off
  TransGearCmd : Outport  Port=3  VectorParamsAs1DForOutWhenUnconnected=off
  TransGear : Outport  Port=4  VectorParamsAs1DForOutWhenUnconnected=off
  DrvShftTrq : Outport  Port=5  VectorParamsAs1DForOutWhenUnconnected=off
  wires:
  Nmtr/1 -> DrvShftTrq/1
  Signal Specification1/1 -> Unit Conversion/1
  Signal Specification/1 -> MtrSpd/1
  "Nmtr "/1 -> Reshape/1
  Unit Conversion/1 -> Signal Specification/1
  GearCmd/1 -> Switch/2
  Mapped Motors/1(MtrTrq) -> MtrTau/1
  MtrTau/1 -> Nmtr/1, Product/2, MtrTrq/1  "MtrTrq"
  HndWhl/1 -> Torque Management/2(HndWhl)
  r/1 -> Saturation/1
  Switch/1 -> TransGearCmd/1, TransGear/1
  "N "/1 -> Switch/3
  D/1 -> Switch/1
  Saturation/1 -> Torque Management/3(r)
  Acc/1 -> Torque Management/1(Acc)
  AxlSpd/1 -> "Nmtr "/1
  Reshape/1 -> Mapped Motors/2(MtrSpd), Product/1, Signal Specification1/1
  Mapped Motors/2(BattCurr) -> Sum of Elements/1  "BattCurr"
  Sum of Elements/1 -> Terminator/1  "TotalBattCurr"
  Product/1 -> 1e-3/1
  1e-3/1 -> Terminator1/1  "MtrPwrkW"
  MATLAB Function/1(V_batt) -> Mapped Motors/1(BattVolt)
  Mapped Motors/3(TrqLimCmd) -> Terminator2/1  "TrqLimCmd"
  MATLAB Function/2(SOC) -> Scope/1
  Torque Management/1(MtrTrqCmd) -> Reshape1/1
  Reshape1/1 -> Mapped Motors/3(TrqCmd)  "TrqCmd"

== system Task 2 – Battery Modeling/Formula Student Vehicle/Simulink Physics - 7DOF/Powertrain & Driveline/Powertrain/ICE Powertrain ==
  Acc : Inport
  GearCmd : Inport  Port=2
  AxlSpd : Inport  Port=3
  Bus Selector : BusSelector  OutputSignals=Trans.TransGearCmd,Trans.TransGear
  Gain1 : Gain  Gain=100
  Powertrain : autolibutils/Cont LPF  wc=10*pi  AbsoluteTolerance=auto  aMode=2
  Signal Specification : SignalSpecification  Unit=rpm
  Simple Engine : autolibsharedmappedengines/Simple Engine  f_tqmax=Eng.Tbts  f_tqmax_n_bpt=Eng.Nbts  Lhv=4.6E+7  Sg=0.754  BsfcAvg=350  aMode=2
      settings: LibrarySourceBlock=vdynlib/Powertrain/Propulsion/Simple Engine
  Terminator : Terminator
  Transmission : Subsystem  Variant=on  VariantControlMode=label  LabelModeActiveChoice=0
  MtrTrq : Outport  VectorParamsAs1DForOutWhenUnconnected=off
  MtrSpd : Outport  Port=2  VectorParamsAs1DForOutWhenUnconnected=off
  TransGearCmd : Outport  Port=3  VectorParamsAs1DForOutWhenUnconnected=off
  TransGear : Outport  Port=4  VectorParamsAs1DForOutWhenUnconnected=off
  DrvShftTrq : Outport  Port=5  VectorParamsAs1DForOutWhenUnconnected=off
  wires:
  Acc/1 -> Gain1/1
  Signal Specification/1 -> Simple Engine/2, MtrSpd/1
  Simple Engine/2 -> Powertrain/1
  Gain1/1 -> Simple Engine/1
  Transmission/1(EngSpd) -> Signal Specification/1
  Simple Engine/1 -> Terminator/1
  Transmission/2(Info) -> Bus Selector/1
  Bus Selector/1 -> TransGearCmd/1  "<TransGearCmd>"
  Bus Selector/2 -> TransGear/1  "<TransGear>"
  GearCmd/1 -> Transmission/2(GearCmd)
  Powertrain/1 -> Transmission/1(EngTrq), MtrTrq/1
  Transmission/3(DrvShfTrq) -> DrvShftTrq/1
  AxlSpd/1 -> Transmission/3(PropShftSpd)

== system Task 2 – Battery Modeling/Visualization/3D Visualization/Enabled/3D Visualization/Disabled ==

== system Task 2 – Battery Modeling/Visualization/3D Visualization/Enabled/3D Visualization/Ground Following ==
  VehFdbk : Inport
  Annotations : Subsystem  Variant=on  VariantControl=Annotations
  Bus Selector3 : BusSelector  OutputSignals=VehFdbk.InertFrm.Cg.Disp.X,VehFdbk.InertFrm.Cg.Disp.Y,VehFdbk.InertFrm.Cg.Ang.psi,Driver.Light controls
  Path : Subsystem  Variant=on  VariantControl=Choice
  Simulation 3D Scene Configuration : sim3dlib/Simulation 3D Scene Configuration  Priority=0  ProjectFormat=Default Scenes  SceneDesc=Open surface  ProjectName=L:\BR2025ad\matlab\toolbox\shared\sim3d_projects\automotive_project_windows\UE\WindowsNoEditor\VehicleSimulation.exe  ScenePath=/Game/Maps/HwStrght  EnableOpenDRIVE=off  vehTagList={'Custom';'GamePhysVehPath';'GrndVehPath';'Scene Origin';'Sim3dActor1';'SimulinkPhysVehPath';'SimulinkVehicle1';'SimulinkVehicle2';'SimulinkVehicle3'}  vehTag=SimulinkVehicle3  AttachedCameraRelativeTranslation=[0 0 0]  FreeCameraDefaultInitialTranslation=[-6, 0, 2]  AttachedCameraRelativeRotation=[0 0 0]  FreeCameraDefaultInitialRotation=[0, -15, 0]  ViewpointName=Custom  FreeCameraInitialTranslation=[0 0 0]  ViewpointTranslation=[0 0 0]  FreeCameraInitialRotation=[0 0 0]  ViewpointRotation=[0 0 0]  OpVisEn=off  Ts=Ts  EnableWindow=on  EnableRemoteAccess=off  EnableWeather=off  SunAzimuth=90  SunAltitude=40.0  EnableGeospatialSun=off  Latitude=0  Longitude=0  Date=2023-01-01  Time=10:30:00  GeoTimeZone=-5.0  SunDaylightSaving=off  wind=1  clouds=10  EnableVolumetricClouds=off  CloudCoverage=0  CloudAltitude=6  fog=0  rain=0  RaindropsEffect=off  SnowDensity=0  EnableGeospatial=off  TilesetSource=Earth terrain  UseTrueOrigin=off  OriginHeight=200  OriginLatitude=40.744652  OriginLongitude=-73.988864  MapStyle=Aerial  AdditionalAssetIDs=[]  UseAdvancedSunSky=off  SolarTime=11  TimeZone=-5  Day=21  Month=9  Year=2022  UseDaylightSavingTime=on  DSTStartDay=10  DSTStartMonth=3  DSTEndDay=3  DSTEndMonth=11  DSTSwitchHour=2  sensorTag=MainCamera1  sensorId=1  sensorName=MainCamera1  mountLoc=Origin  offsetFlag=off  tmountOffset=[0, 0, 0]  rmountOffset=[0, 0, 0]  HorizontalResolution=1280  VerticalResolution=720  HorizontalFOV=60  mountPoint=[0 0 0]  mountOrientation=[0 0 0]  aMode=2  ID=1  GeoTrigger=Inactive  ViewNameList={'Custom'}  ViewTranslationList={'[0 0 0]'}  ViewRotationList={'[0 0 0]'}
      settings: LibrarySourceBlock=vdynlib/Vehicle Scenarios/Sim3D/Sim3D Core/Simulation 3D Scene Configuration
  Simulation 3D Vehicle with Ground Following : sim3dautolib/Simulation 3D Vehicle with Ground Following VDBS  Priority=-1  PassVehMesh=Hatchback  MeshPath=/MathWorksSimulation/Vehicles/Muscle/Meshes/SK_MuscleCar.SK_MuscleCar  TrackWidth=1.9  WheelBase=3  WheelRadius=0.35  VehColor=Red  CoordinateSystem=SAE  InitialPos=[ VEH.InitialLongPosition, VEH.InitialLatPosition, VEH.InitialVertPosition ]  InitialRot=[VEH.InitialRollAngle VEH.InitialPitchAngle VEH.InitialYawAngle]  ActorName=SimulinkVehicle3  VehLightsControl=on  HeadlightColor=[ 1, 1, 1 ]  HighBeamIntensity=100000  LowBeamIntensity=60000  HighBeamConeAngle=1.22  LowBeamConeAngle=1.22  LeftHeadlightOrientation=[ 0, 0 ]  RightHeadlightOrientation=[ 0, 0 ]  BrakelightIntensity=200  ReverselightIntensity=500  SignallightIntensity=500  SignallightPeriod=1  SignalPulseWidth=50  SampleTime=Ts  ActorType=SimulinkVehicle  ID=3  aMode=2  ActorTag=SimulinkVehicle3  CoordinateScheme=SAE
      settings: LibrarySourceBlock=vehdynlibsim3d/Simulation 3D Vehicle with Ground Following
  wires:
  Bus Selector3/1 -> Simulation 3D Vehicle with Ground Following/1  "<X>"
  VehFdbk/1 -> Path/1(VehFdbk), Annotations/1(VehFdbk), Bus Selector3/1
  Bus Selector3/2 -> Simulation 3D Vehicle with Ground Following/2  "<Y>"
  Bus Selector3/4 -> Simulation 3D Vehicle with Ground Following/4  "<Light controls>"
  Bus Selector3/3 -> Simulation 3D Vehicle with Ground Following/3  "<psi>"
